simulink model "hopper_6dof"  (R2025a)
settings: Solver=VariableStepAuto  StartTime=0.0  StopTime=10  RelTol=1e-3
values from neighbouring files (symbols this model uses):
  AVI = size_avionics(IN)    [main.m]
  bp = data(:,1)    [load_lookup.m]
  ENGINE = size_engine(IN)    [main.m]
  IN = mission_inputs()    [main.m]
  OUT = Outputs(IN, VEH, TANKS, STRUCT)    [main.m]
  TANKS = size_tanks(IN)    [main.m]
  tbl1 = data(:,2)    [load_lookup.m]
  tbl2 = data(:,3)    [load_lookup.m]
libraries: dspindex x1, aerolibanim x1
settings Model: Creator=asing  LastModifiedBy=asing

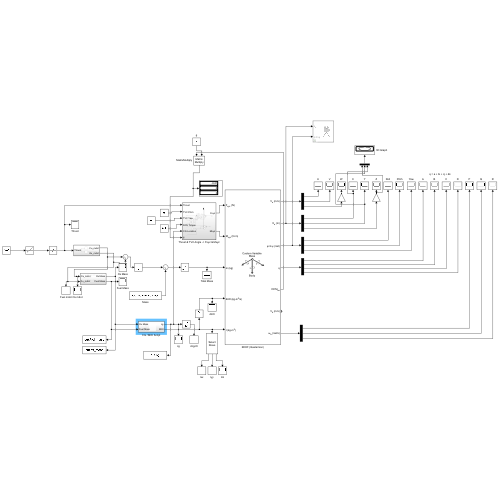
[thumbnail: Simulink's stored preview of the top-level diagram]
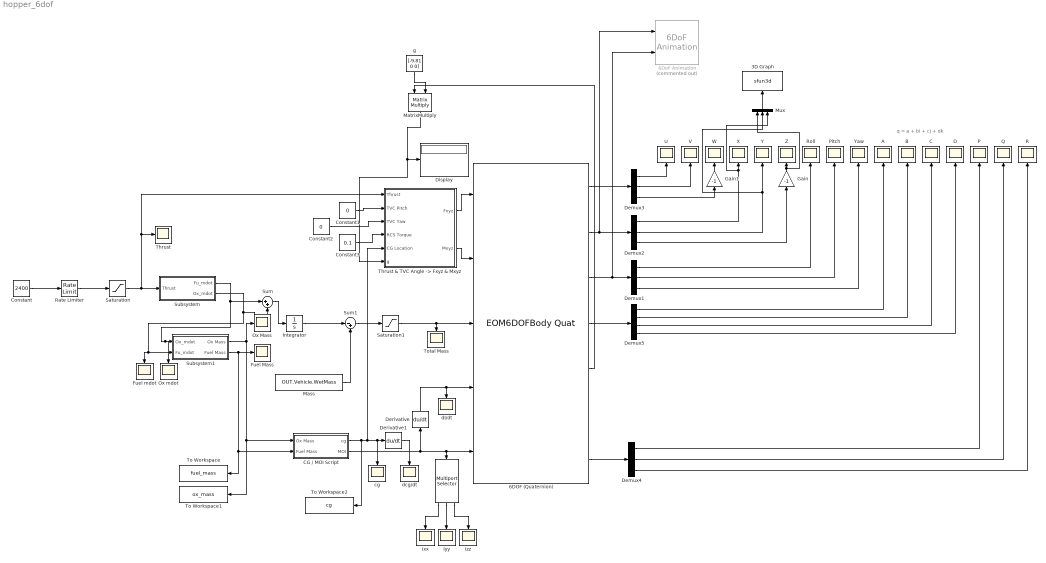
== system hopper_6dof ==
  note: q = a + bi + cj + dk
  " " : dspindex/Multiport Selector  rowsOrCols=Rows  idxCellArray={1,2,3}  idxErrMode=Clip Index
      settings: LibrarySourceBlock=|
      | dsphdlsupportsigmgmt/Multiport
      | Selector
  3D Graph : S-Function  LoadFcn=if exist('sfun3d','file'), sfun3d([],[],[],'LoadBlock'); end  FunctionName=sfun3d  Parameters=ax,T,np,cp,gd,ls,mk,mx,hd,tb  SFunctionDeploymentMode=off  EnableBusSupport=off  mask(3D Graph){np=1, ax=[-50 50 -50 50 -50 50], mx=1e4, T=0.1, cp=[15 30 5], gd=on, hd=off, tb=off, ls=-, mk=none}
      mask prompts: np "Number of moving points (lines)"; ax "Range: [xmin xmax  ymin ymax zmin zmax]"; mx "Max number of points in each line"; T "Sampling Time"; cp "Camera position (use [0 0 1] for 2D XY view)"; gd "Grid (on|off)"; hd "HeadMarkers (on|off)"; tb "Toolbar (on|off)"; ls "LineStyle"; mk "LineMarker"
      mask help:
      | This block plots the position of several points in the XYZ space. The input contains the coordinates of all the points (x1,y1,z1,x2,y2,z2,...).
      | The number of moving points (lines), the XYZ ranges, sampling time, camera position, and grid (among other things) can be set as mask parameters.
      settings: CopyFcn=if exist('sfun3d','file'), sfun3d([],[],[],'CopyBlock'); end  DeleteFcn=if exist('sfun3d','file'), sfun3d([],[],[],'DeleteBlock'); end  NameChangeFcn=if exist('sfun3d','file'), sfun3d([],[],[],'NameChange'); end
      mask Help:
      | This block plots the position of several points in the XYZ space. The input contains the coordinates of all the points (x1,y1,z1,x2,y2,z2,...).
      | The number of moving points (lines), the XYZ ranges, sampling time, camera position, and grid (among other things) can be set as mask parameters.
      mask TypeOptions ls: - | -- | : | -. | none
      mask TypeOptions mk: none | . | + | o | * | x | square | diamond | v | ^ | > | < | pentagram | hexagram
      mask Display: plot([.05 .95 .95 .05 .05],[.45 .45 .95 .95 .45], 0.5+cos(0:0.1:2*pi)*0.3,0.7+sin(0:0.1:2*pi)*0.2)
  6DOF (Quaternion) : EOM6DOFBodyQuat  mtype=Custom Variable
  6DoF Animation : aerolibanim/6DoF Animation  Commented=on  u1=[0 4000 -2000 2000 -5000 -3000]  u2=0.1  u3=1.0  u4=[4000 0 -5000]  u5=Fly alongside  u6=[2000 500 -3150]  u7=10  u8=on
  A : Scope
      settings: ActiveDisplayYMinimum=-1  ActiveDisplayYMaximum=1  DataLoggingVariableName=ScopeData12
  B : Scope
      settings: ActiveDisplayYMinimum=-1  ActiveDisplayYMaximum=1  DataLoggingVariableName=ScopeData13
  C : Scope
      settings: DataLoggingVariableName=ScopeData14
  CG / MOI Script : Subsystem
  Constant : Constant  Value=2400
  Constant1 : Constant  Value=0
  Constant2 : Constant  Value=0
  Constant3 : Constant  Value=0.1
  D : Scope
      settings: DataLoggingVariableName=ScopeData15
  Demux{1..4} (4 alike) : Demux  Outputs=3
  Demux5 : Demux
  Derivative : Derivative
  Derivative1 : Derivative
  Display : Display
  Fuel Mass : Scope
      settings: ActiveDisplayYMinimum=-1  ActiveDisplayYMaximum=1  DataLoggingVariableName=ScopeData18
  Fuel mdot : Scope
      settings: DataLoggingVariableName=ScopeData20
  Gain : Gain  Gain=-1
  Gain1 : Gain  Gain=-1
  Integrator : Integrator
  Ixx : Scope
      settings: ActiveDisplayYMinimum=-0.048827148723178677  ActiveDisplayYMaximum=0.4394443385086082  DataLoggingVariableName=ScopeData21
  Iyy : Scope
      settings: ActiveDisplayYMinimum=-1  ActiveDisplayYMaximum=1  DataLoggingVariableName=ScopeData26
  Izz : Scope
      settings: ActiveDisplayYMinimum=-2.8210574648941242  ActiveDisplayYMaximum=25.389517184047122  DataLoggingVariableName=ScopeData27
  Mass : Constant  Value=OUT.Vehicle.WetMass
  MatrixMultiply : Product  Multiplication=Matrix(*)
  Mux : Mux  Inputs=3
  Ox Mass : Scope
      settings: ActiveDisplayYMinimum=-1  ActiveDisplayYMaximum=1  DataLoggingVariableName=ScopeData17
  Ox mdot : Scope
      settings: ActiveDisplayYMinimum=-1  ActiveDisplayYMaximum=1  DataLoggingVariableName=ScopeData19
  P : Scope
      settings: ActiveDisplayYMinimum=-1  ActiveDisplayYMaximum=1  DataLoggingVariableName=ScopeData9
  Pitch : Scope
      settings: ActiveDisplayYMinimum=-0.98149890313936494  ActiveDisplayYMaximum=0.98171603037850841  DataLoggingVariableName=ScopeData4
  Q : Scope
      settings: ActiveDisplayYMinimum=-1  ActiveDisplayYMaximum=1  DataLoggingVariableName=ScopeData10
  R : Scope
      settings: ActiveDisplayYMinimum=-1  ActiveDisplayYMaximum=1  DataLoggingVariableName=ScopeData11
  Rate Limiter : RateLimiter  RisingSlewLimit=500  FallingSlewLimit=-500  SampleTimeMode=inherited
  Roll : Scope
      settings: ActiveDisplayYMinimum=-3.9220611360258721  ActiveDisplayYMaximum=3.9240500621746381  DataLoggingVariableName=ScopeData3
  Saturation : Saturate  UpperLimit=2400  LowerLimit=890
  Saturation1 : Saturate  UpperLimit=OUT.Vehicle.WetMass  LowerLimit=OUT.Vehicle.DryMass
  Subsystem : Subsystem
  Subsystem1 : Subsystem
  Sum : Sum  Inputs=|++
  Sum1 : Sum  Inputs=|-+
  Thrust : Scope
      settings: ActiveDisplayYMinimum=-1  ActiveDisplayYMaximum=1  DataLoggingVariableName=ScopeData25
  "Thrust & TVC Angle -> Fxyz & Mxyz" : Subsystem
  To Workspace : ToWorkspace  VariableName=fuel_mass  SaveFormat=Timeseries  SampleTime=-1
  To Workspace1 : ToWorkspace  VariableName=ox_mass  SaveFormat=Timeseries  SampleTime=-1
  To Workspace2 : ToWorkspace  VariableName=cg  SaveFormat=Timeseries  SampleTime=-1
  Total Mass : Scope
      settings: ActiveDisplayYMinimum=99.969777000507577  ActiveDisplayYMaximum=116.79899243992762  DataLoggingVariableName=ScopeData16
  U : Scope
      settings: DataLoggingVariableName=ScopeData6
  V : Scope
      settings: DataLoggingVariableName=ScopeData7
  W : Scope
      settings: DataLoggingVariableName=ScopeData8
  X : Scope
      settings: ActiveDisplayYMinimum=-1  ActiveDisplayYMaximum=1
  Y : Scope
      settings: ActiveDisplayYMinimum=-235.33662889488539  ActiveDisplayYMaximum=201.09811638610955
  Yaw : Scope
      settings: ActiveDisplayYMinimum=-3.5399153182965852  ActiveDisplayYMaximum=4.3139775267714358  DataLoggingVariableName=ScopeData5
  Z : Scope
      settings: ActiveDisplayYMinimum=-1  ActiveDisplayYMaximum=1  DataLoggingVariableName=ScopeData2
  cg : Scope
      settings: ActiveDisplayYMinimum=1.0809554570779685  ActiveDisplayYMaximum=1.1447531542625193  DataLoggingVariableName=ScopeData23
  dI/dt : Scope
      settings: ActiveDisplayYMinimum=-5.4952195596838944  ActiveDisplayYMaximum=2.8768789367976191  DataLoggingVariableName=ScopeData22
  dcg/dt : Scope
      settings: DataLoggingVariableName=ScopeData24
  g : Constant  Value=[-9.81 0 0]
  wires:
  6DOF (Quaternion)/2 -> 6DoF Animation/1, Demux2/1
  6DOF (Quaternion)/3 -> 6DoF Animation/2, Demux1/1
  Demux2/1 -> Mux/3, X/1
  Demux2/2 -> Y/1, Mux/2
  Demux2/3 -> Gain/1
  Gain/1 -> Mux/1, Z/1
  Demux1/1 -> Roll/1
  Demux1/2 -> Pitch/1
  Demux1/3 -> Yaw/1
  6DOF (Quaternion)/1 -> Demux3/1
  Demux3/1 -> U/1
  Demux3/2 -> V/1
  Demux3/3 -> Gain1/1
  6DOF (Quaternion)/4 -> Demux5/1
  6DOF (Quaternion)/7 -> Demux4/1
  Demux4/1 -> P/1
  Demux4/2 -> Q/1
  Demux4/3 -> R/1
  Demux5/1 -> A/1
  Demux5/2 -> B/1
  Demux5/3 -> C/1
  Demux5/4 -> D/1
  Gain1/1 -> W/1
  Subsystem/1(Fu_mdot) -> Ox mdot/1, Subsystem1/1(Ox_mdot), Sum/1
  Subsystem/2(Ox_mdot) -> Fuel mdot/1, Subsystem1/2(Fu_mdot), Sum/2
  Sum/1 -> Integrator/1
  Integrator/1 -> Sum1/1
  Mass/1 -> Sum1/2
  Sum1/1 -> Saturation1/1
  Saturation1/1 -> Total Mass/1, 6DOF (Quaternion)/3
  Subsystem1/1(Ox Mass) -> To Workspace1/1, CG / MOI Script/1(Ox Mass), Ox Mass/1
  Subsystem1/2(Fuel Mass) -> Fuel Mass/1, To Workspace/1, CG / MOI Script/2(Fuel Mass)
  CG / MOI Script/2(MOI) -> Derivative/1, 6DOF (Quaternion)/5, " "/1
  Derivative/1 -> 6DOF (Quaternion)/4, dI/dt/1
  CG / MOI Script/1(cg) -> To Workspace2/1, Derivative1/1, cg/1, "Thrust & TVC Angle -> Fxyz & Mxyz"/5(CG Location)
  Derivative1/1 -> dcg/dt/1
  "Thrust & TVC Angle -> Fxyz & Mxyz"/1(Fxyz) -> 6DOF (Quaternion)/1
  "Thrust & TVC Angle -> Fxyz & Mxyz"/2(Mxyz) -> 6DOF (Quaternion)/2
  Rate Limiter/1 -> Saturation/1
  Saturation/1 -> Subsystem/1(Thrust), Thrust/1, "Thrust & TVC Angle -> Fxyz & Mxyz"/1("Thrust ")
  Constant/1 -> Rate Limiter/1
  Constant1/1 -> "Thrust & TVC Angle -> Fxyz & Mxyz"/2(TVC Pitch)
  Constant2/1 -> "Thrust & TVC Angle -> Fxyz & Mxyz"/3(TVC Yaw)
  Constant3/1 -> "Thrust & TVC Angle -> Fxyz & Mxyz"/4(RCS Torque)
  " "/1 -> Ixx/1
  " "/2 -> Iyy/1
  " "/3 -> Izz/1
  Mux/1 -> 3D Graph/1
  g/1 -> MatrixMultiply/2
  6DOF (Quaternion)/5 -> MatrixMultiply/1
  MatrixMultiply/1 -> "Thrust & TVC Angle -> Fxyz & Mxyz"/6(g), Display/1

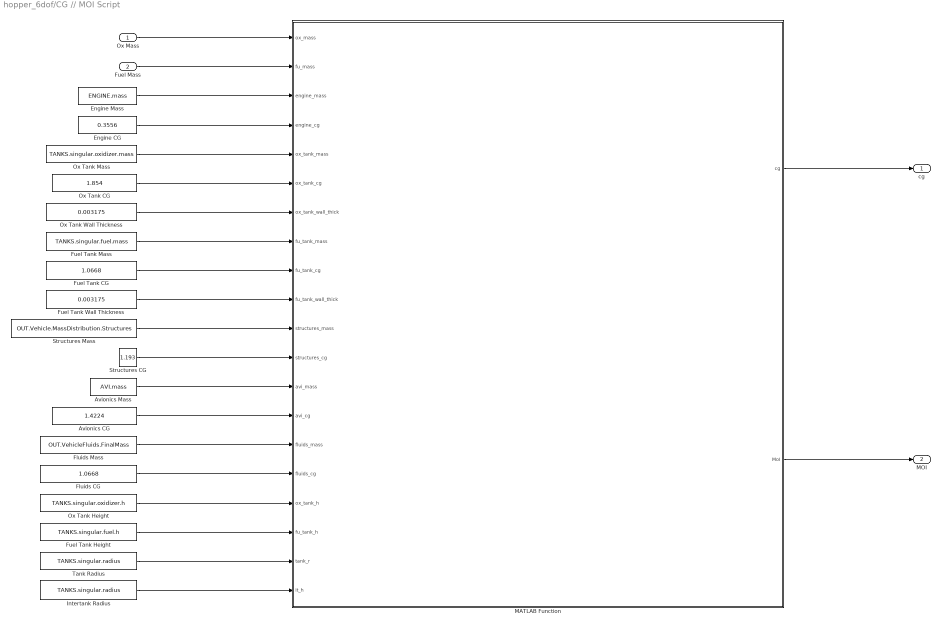
== system hopper_6dof/CG // MOI Script ==
  Ox Mass : Inport
  Fuel Mass : Inport  Port=2
  Avionics CG : Constant  Value=1.4224
  Avionics Mass : Constant  Value=AVI.mass
  Engine CG : Constant  Value=0.3556
  Engine Mass : Constant  Value=ENGINE.mass
  Fluids CG : Constant  Value=1.0668
  Fluids Mass : Constant  Value=OUT.VehicleFluids.FinalMass
  Fuel Tank CG : Constant  Value=1.0668
  Fuel Tank Height : Constant  Value=TANKS.singular.fuel.h
  Fuel Tank Mass : Constant  Value=TANKS.singular.fuel.mass
  Fuel Tank Wall Thickness : Constant  Value=0.003175
  Intertank Radius : Constant  Value=TANKS.singular.radius
  MATLAB Function : MATLAB Function  TreatAsAtomicUnit=on
  Ox Tank CG : Constant  Value=1.854
  Ox Tank Height : Constant  Value=TANKS.singular.oxidizer.h
  Ox Tank Mass : Constant  Value=TANKS.singular.oxidizer.mass
  Ox Tank Wall Thickness : Constant  Value=0.003175
  Structures CG : Constant  Value=1.193
  Structures Mass : Constant  Value=OUT.Vehicle.MassDistribution.Structures
  Tank Radius : Constant  Value=TANKS.singular.radius
  cg : Outport
  MOI : Outport  Port=2
  wires:
  Ox Mass/1 -> MATLAB Function/1(ox_mass)
  Fuel Mass/1 -> MATLAB Function/2(fu_mass)
  Engine Mass/1 -> MATLAB Function/3(engine_mass)
  Engine CG/1 -> MATLAB Function/4(engine_cg)
  Ox Tank Mass/1 -> MATLAB Function/5(ox_tank_mass)
  Ox Tank CG/1 -> MATLAB Function/6(ox_tank_cg)
  Ox Tank Wall Thickness/1 -> MATLAB Function/7(ox_tank_wall_thick)
  Fuel Tank Mass/1 -> MATLAB Function/8(fu_tank_mass)
  Fuel Tank CG/1 -> MATLAB Function/9(fu_tank_cg)
  Fuel Tank Wall Thickness/1 -> MATLAB Function/10(fu_tank_wall_thick)
  Structures Mass/1 -> MATLAB Function/11(structures_mass)
  Structures CG/1 -> MATLAB Function/12(structures_cg)
  Avionics Mass/1 -> MATLAB Function/13(avi_mass)
  Avionics CG/1 -> MATLAB Function/14(avi_cg)
  Fluids Mass/1 -> MATLAB Function/15(fluids_mass)
  Fluids CG/1 -> MATLAB Function/16(fluids_cg)
  Ox Tank Height/1 -> MATLAB Function/17(ox_tank_h)
  Fuel Tank Height/1 -> MATLAB Function/18(fu_tank_h)
  Tank Radius/1 -> MATLAB Function/19(tank_r)
  Intertank Radius/1 -> MATLAB Function/20(it_h)
  MATLAB Function/2(MoI) -> MOI/1
  MATLAB Function/1(cg) -> cg/1

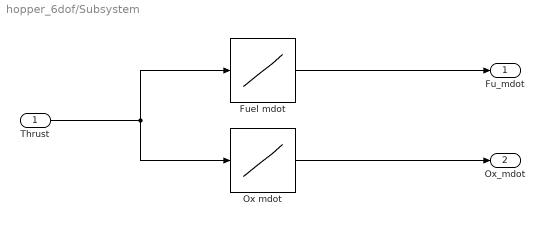
== system hopper_6dof/Subsystem ==
  Thrust : Inport
  Fuel mdot : Lookup_n-D  NumberOfTableDimensions=1  BreakpointsForDimension1=bp  Table=tbl2  InternalRulePriority=Speed  RndMeth=Simplest
  Ox mdot : Lookup_n-D  NumberOfTableDimensions=1  BreakpointsForDimension1=bp  Table=tbl1  InternalRulePriority=Speed  RndMeth=Simplest
  Fu_mdot : Outport
  Ox_mdot : Outport  Port=2
  wires:
  Thrust/1 -> Ox mdot/1, Fuel mdot/1
  Fuel mdot/1 -> Fu_mdot/1
  Ox mdot/1 -> Ox_mdot/1

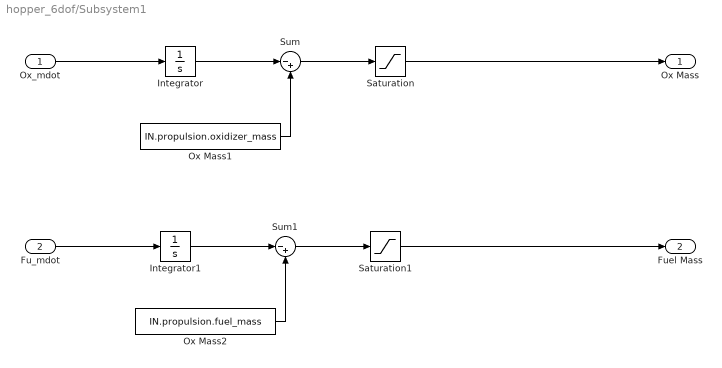
== system hopper_6dof/Subsystem1 ==
  Ox_mdot : Inport
  Fu_mdot : Inport  Port=2
  Integrator : Integrator
  Integrator1 : Integrator
  Ox Mass1 : Constant  Value=IN.propulsion.oxidizer_mass
  Ox Mass2 : Constant  Value=IN.propulsion.fuel_mass
  Saturation : Saturate  UpperLimit=IN.propulsion.oxidizer_mass  LowerLimit=0
  Saturation1 : Saturate  UpperLimit=IN.propulsion.fuel_mass  LowerLimit=0
  Sum : Sum  Inputs=|-+
  Sum1 : Sum  Inputs=|-+
  Ox Mass : Outport
  Fuel Mass : Outport  Port=2
  wires:
  Ox_mdot/1 -> Integrator/1
  Integrator/1 -> Sum/1
  Ox Mass1/1 -> Sum/2
  Sum/1 -> Saturation/1
  Saturation/1 -> Ox Mass/1
  Sum1/1 -> Saturation1/1
  Saturation1/1 -> Fuel Mass/1
  Fu_mdot/1 -> Integrator1/1
  Ox Mass2/1 -> Sum1/2
  Integrator1/1 -> Sum1/1

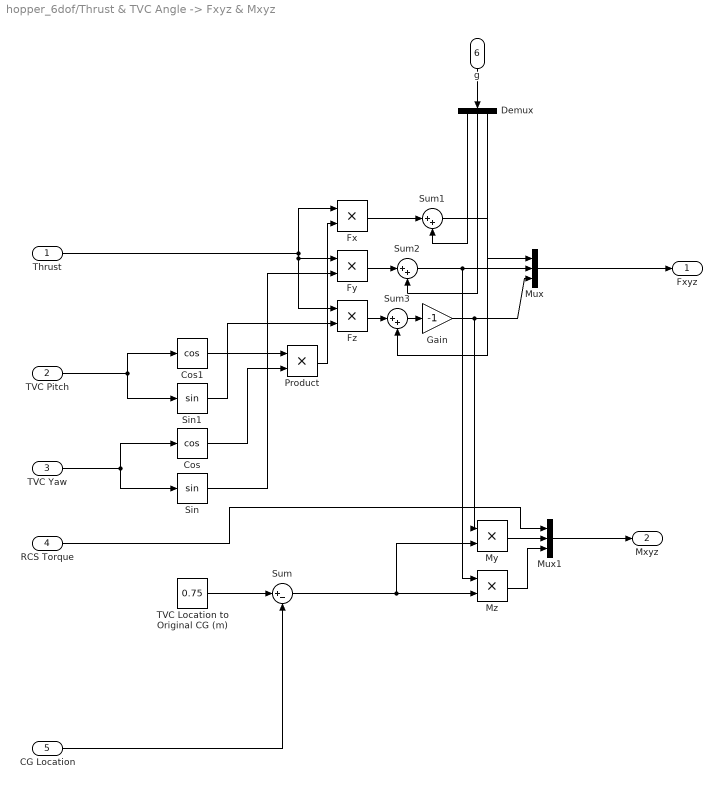
== system hopper_6dof/Thrust & TVC Angle -> Fxyz & Mxyz ==
  "Thrust " : Inport
  TVC Pitch : Inport  Port=2
  TVC Yaw : Inport  Port=3
  RCS Torque : Inport  Port=4
  CG Location : Inport  Port=5
  g : Inport  Port=6
  Cos : Trigonometry  Operator=cos
  Cos1 : Trigonometry  Operator=cos
  Demux : Demux  Outputs=3
  Fx : Product
  Fy : Product
  Fz : Product
  Gain : Gain  Gain=-1
  Mux : Mux  Inputs=3
  Mux1 : Mux  Inputs=3
  My : Product
  Mz : Product
  Product : Product
  Sin : Trigonometry
  Sin1 : Trigonometry
  Sum : Sum  Inputs=|+-
  Sum1 : Sum  Inputs=|++
  Sum2 : Sum  Inputs=|++
  Sum3 : Sum  Inputs=|++
  TVC Location to Original CG (m) : Constant  Value=0.75
  Fxyz : Outport
  Mxyz : Outport  Port=2
  wires:
  TVC Yaw/1 -> Sin/1, Cos/1
  TVC Pitch/1 -> Sin1/1, Cos1/1
  Cos1/1 -> Product/1
  Cos/1 -> Product/2
  Product/1 -> Fx/2
  "Thrust "/1 -> Fy/1, Fz/1, Fx/1
  Sin/1 -> Fy/2
  Sin1/1 -> Fz/2
  Mux/1 -> Fxyz/1
  TVC Location to Original CG (m)/1 -> Sum/1
  CG Location/1 -> Sum/2
  Sum/1 -> My/2, Mz/2
  RCS Torque/1 -> Mux1/1
  My/1 -> Mux1/2
  Mz/1 -> Mux1/3
  Mux1/1 -> Mxyz/1
  Gain/1 -> Mux/3, My/1
  Fx/1 -> Sum1/1
  Sum1/1 -> Mux/1
  g/1 -> Demux/1
  Demux/1 -> Sum1/2
  Fy/1 -> Sum2/1
  Sum2/1 -> Mz/1, Mux/2
  Fz/1 -> Sum3/1
  Sum3/1 -> Gain/1
  Demux/2 -> Sum2/2
  Demux/3 -> Sum3/2

== matlab function hopper_6dof/CG // MOI Script/MATLAB Function ==
  data: ox_mass input; cg output; fu_mass input; engine_mass input; engine_cg input; ox_tank_mass input; ox_tank_cg input; ox_tank_wall_thick input; fu_tank_mass input; fu_tank_cg input; fu_tank_wall_thick input; structures_mass input; structures_cg input; avi_mass input; avi_cg input; fluids_mass input; fluids_cg input; ox_tank_h input; fu_tank_h input; tank_r input; it_h input; MoI output
function [cg, MoI] = cg_sim(ox_mass, fu_mass, engine_mass, engine_cg, ox_tank_mass, ox_tank_cg, ox_tank_wall_thick, fu_tank_mass, fu_tank_cg, fu_tank_wall_thick, structures_mass, structures_cg, avi_mass, avi_cg, fluids_mass, fluids_cg, ox_tank_h, fu_tank_h, tank_r, it_h)
%CG_SIM Calculates the Center of Gravity and Moment of Inertia Matrix
%   Inputs are masses (kg), CG positions (m), and dimensions (m).

    %% 1. Constants and Unit Conversions
        ox_density = 1141;   % kg/m^3
        fu_density = 800;    % kg/m^3
    al_density = 2700;   % kg/m^3 (Density of Al6061)
    
    % Engine dimensions: 4 inch radius, 1 ft length
    eng_r = 4 * 0.0254;  % inches to meters
    eng_h = 1 * 0.3048;  % ft to meters

    %% 2. End Cap Geometry & Mass (NEW)
    % Modeled as solid cylinders attached to the ends of the tank shells.
    % Height of cap = wall thickness of the respective tank.
    
    % --- Oxidizer Tank Caps ---
    h_ox_cap = ox_tank_wall_thick;
    vol_ox_cap = pi * tank_r^2 * h_ox_cap;
    m_ox_cap   = al_density * vol_ox_cap; % Mass of ONE cap
    
    % Positions (Top and Bottom of the hollow shell)
    % Z = Tank_CG +/- (Tank_H/2 + Cap_H/2)
    z_ox_cap_bot = ox_tank_cg - (ox_tank_h / 2) - (h_ox_cap / 2);
    z_ox_cap_top = ox_tank_cg + (ox_tank_h / 2) + (h_ox_cap / 2);

    % --- Fuel Tank Caps ---
    h_fu_cap = fu_tank_wall_thick;
    vol_fu_cap = pi * tank_r^2 * h_fu_cap;
    m_fu_cap   = al_density * vol_fu_cap; % Mass of ONE cap
    
    % Positions
    z_fu_cap_bot = fu_tank_cg - (fu_tank_h / 2) - (h_fu_cap / 2);
    z_fu_cap_top = fu_tank_cg + (fu_tank_h / 2) + (h_fu_cap / 2);

    %% 3. Fluid Geometry Calculations
    % Fuel Fluid
    if fu_mass > 0
        h_fu_fluid = (fu_mass / fu_density) / (pi * tank_r^2);
        % Fluid sits at the bottom of the tank shell
        z_fu_fluid = (fu_tank_cg - fu_tank_h/2) + (h_fu_fluid / 2);
    else
        h_fu_fluid = 0; z_fu_fluid = 0;
    end

    % Oxidizer Fluid
    if ox_mass > 0
        h_ox_fluid = (ox_mass / ox_density) / (pi * tank_r^2);
        z_ox_fluid = (ox_tank_cg - ox_tank_h/2) + (h_ox_fluid / 2);
    else
        h_ox_fluid = 0; z_ox_fluid = 0;
    end

    %% 4. Calculate System Center of Gravity (CG)
    % Sum of Moments = sum(mass * position)
    moment_sum = ...
        engine_mass * engine_cg + ...
        fu_tank_mass * fu_tank_cg + ...
        ox_tank_mass * ox_tank_cg + ...
        structures_mass * structures_cg + ...
        avi_mass * avi_cg + ...
        fu_mass * z_fu_fluid + ...
        ox_mass * z_ox_fluid + ...
        m_ox_cap * z_ox_cap_bot + ... 
        m_ox_cap * z_ox_cap_top + ...  
        m_fu_cap * z_fu_cap_bot + ...  
        m_fu_cap * z_fu_cap_top;      

    total_mass = engine_mass + fu_tank_mass + ox_tank_mass + ...
                 structures_mass + avi_mass + fu_mass + ox_mass + ...
                 2 * m_ox_cap + 2 * m_fu_cap;

    if total_mass > 0
        cg = moment_sum / total_mass; % return 1
    else
        cg = 0;
    end

    %% 5. Calculate Moments of Inertia (MoI)
    % Anonymous functions for inertia - shout out gemini for this one
    calc_solid_Izz = @(m, r) 0.5 * m * r^2;
    calc_solid_Ixx = @(m, r, h) (1/12) * m * (3*r^2 + h^2);
    calc_hollow_Izz = @(m, ro, ri) 0.5 * m * (ro^2 + ri^2);
    calc_hollow_Ixx = @(m, ro, ri, h) (1/12) * m * (3*(ro^2 + ri^2) + h^2);

    % --- A. Engine ---
    Izz_eng = calc_solid_Izz(engine_mass, eng_r);
    Ixx_eng = calc_solid_Ixx(engine_mass, eng_r, eng_h) + engine_mass * (engine_cg - cg)^2;

    % --- B. Fuel Tank (Hollow Shell) ---
    r_in_fu = tank_r - fu_tank_wall_thick;
    Izz_fut = calc_hollow_Izz(fu_tank_mass, tank_r, r_in_fu);
    Ixx_fut = calc_hollow_Ixx(fu_tank_mass, tank_r, r_in_fu, fu_tank_h) + fu_tank_mass * (fu_tank_cg - cg)^2;

    % --- C. Oxidizer Tank (Hollow Shell) ---
    r_in_ox = tank_r - ox_tank_wall_thick;
    Izz_oxt = calc_hollow_Izz(ox_tank_mass, tank_r, r_in_ox);
    Ixx_oxt = calc_hollow_Ixx(ox_tank_mass, tank_r, r_in_ox, ox_tank_h) + ox_tank_mass * (ox_tank_cg - cg)^2;

    % --- D. Structures --- just asssume cylinder in it
    Izz_str = calc_solid_Izz(structures_mass, tank_r);
    Ixx_str = calc_solid_Ixx(structures_mass, tank_r, it_h) + structures_mass * (structures_cg - cg)^2;

    % --- E. Avionics --- just asssume cylinder in it
    Izz_avi = calc_solid_Izz(avi_mass, tank_r);
    Ixx_avi = calc_solid_Ixx(avi_mass, tank_r, it_h) + avi_mass * (avi_cg - cg)^2;

    % --- F. Fluids ---
    if fu_mass > 0
        Izz_fuf = calc_solid_Izz(fu_mass, tank_r);
        Ixx_fuf = calc_solid_Ixx(fu_mass, tank_r, h_fu_fluid) + fu_mass * (z_fu_fluid - cg)^2;
    else
        Izz_fuf = 0; Ixx_fuf = 0;
    end

    if ox_mass > 0
        Izz_oxf = calc_solid_Izz(ox_mass, tank_r);
        Ixx_oxf = calc_solid_Ixx(ox_mass, tank_r, h_ox_fluid) + ox_mass * (z_ox_fluid - cg)^2;
    else
        Izz_oxf = 0; Ixx_oxf = 0;
    end

    % --- G. End Caps ---
    % 1. Ox Caps (Solid Cylinders)
    % Izz is same for both
    Izz_ox_cap = calc_solid_Izz(m_ox_cap, tank_r);
    Ixx_ox_cap_local = calc_solid_Ixx(m_ox_cap, tank_r, h_ox_cap);
    
    Ixx_ox_caps_total = ...
        (Ixx_ox_cap_local + m_ox_cap * (z_ox_cap_bot - cg)^2) + ... % Bottom Cap
        (Ixx_ox_cap_local + m_ox_cap * (z_ox_cap_top - cg)^2);      % Top Cap

    % 2. Fuel Caps (Solid Cylinders)
    Izz_fu_cap = calc_solid_Izz(m_fu_cap, tank_r);
    Ixx_fu_cap_local = calc_solid_Ixx(m_fu_cap, tank_r, h_fu_cap);
    
    Ixx_fu_caps_total = ...
        (Ixx_fu_cap_local + m_fu_cap * (z_fu_cap_bot - cg)^2) + ... % Bottom Cap
        (Ixx_fu_cap_local + m_fu_cap * (z_fu_cap_top - cg)^2);      % Top Cap

    %% 6. Summation
    Izz_total = Izz_eng + Izz_fut + Izz_oxt + Izz_str + Izz_avi + ...
                Izz_fuf + Izz_oxf + ...
                2*Izz_ox_cap + 2*Izz_fu_cap;
                
    Ixx_total = Ixx_eng + Ixx_fut + Ixx_oxt + Ixx_str + Ixx_avi + ...
                Ixx_fuf + Ixx_oxf + ...
                Ixx_ox_caps_total + Ixx_fu_caps_total;
    
    Iyy_total = Ixx_total; % Symmetry

    MoI = [Izz_total, 0, 0; 
           0, Iyy_total, 0; 
           0, 0, Ixx_total]; % return 2
end
